simulink model "turbo_controller"  (R2025a)
settings: Solver=FixedStepAuto  StartTime=0.0  StopTime=inf  FixedStep=0.001  RelTol=1e-3
PostLoadFcn:
  | % 自动定位同目录CubeMX文件；不需要外部初始化脚本。
  | codertarget.data.setParameterValue('turbo_controller','STM32CubeMX.ProjectFile',fullfile(fileparts(get_param('turbo_controller','FileName')),'turbo_f407.ioc'));
InitFcn:
  | % 中文说明：按原控制器字段与类型创建三组接口总线；控制参数已内嵌。
  | tc_names=["EValve_Cycle" "EValve_Open" "Eblast_Cycle" "Eblast_Open" "Motor_Cycle" "Motor_Open" "EValve_Enable" "Eblast_Enable" "Motor_Enable" "SWO_Firework" "SWO_BleedAir" "EngineState" "Flag_ECUReset_Clear" "Flag_ECUReset_Save" "Flag_Reset_Enable" "Accelerator" "Nc_dem" "Nc"]; tc_types=["uint16" "uint16" "uint16" "uint16" "uint16" "uint16" "uint8" "uint8" "uint8" "uint8" "uint8" "uint8" "uint8" "uint8" "uint8" "single" "single" "single"];
  | for tc_k=1:numel(tc_names)
  |  tc_e(tc_k)=Simulink.BusElement; tc_e(tc_k).Name=char(tc_names(tc_k)); tc_e(tc_k).DataType=char(tc_types(tc_k));
  | end
  | EngineControl_Out=Simulink.Bus; EngineControl_Out.DataScope='Exported'; EngineControl_Out.Elements=tc_e;
  | clear tc_e tc_names tc_types tc_k
  | tc_names=["savedata1" "savedata2" "savedata3" "savedata4" "savedata5" "savedata6" "savedata7" "savedata8" "savedata9" "savedata10" "savedata11" "savedata12" "savedata13" "savedata14" "savedata15" "savedata16" "savedata17" "savedata18" "savedata19" "savedata20" "savedata21" "savedata22" "savedata23" "savedata24" "savedata25"]; tc_types=["single" "single" "single" "single" "single" "single" "single" "single" "single" "single" "single" "single" "single" "single" "single" "single" "single" "single" "single" "single" "single" "single" "single" "single" "single"];
  | for tc_k=1:numel(tc_names)
  |  tc_e(tc_k)=Simulink.BusElement; tc_e(tc_k).Name=char(tc_names(tc_k)); tc_e(tc_k).DataType=char(tc_types(tc_k));
  | end
  | SaveData_Out=Simulink.Bus; SaveData_Out.DataScope='Exported'; SaveData_Out.Elements=tc_e;
  | clear tc_e tc_names tc_types tc_k
  | tc_names=["senddata1" "senddata2" "senddata3" "senddata4" "senddata5" "senddata6" "senddata7" "senddata8" "senddata9" "senddata10" "senddata11" "senddata12" "senddata13" "senddata14" "senddata15" "senddata16" "senddata17" "senddata18" "senddata19" "senddata20" "senddata21" "senddata22" "senddata23" "senddata24" "senddata25" "senddata26" "senddata27" "senddata28" "senddata29"]; tc_types=["uint8" "uint8" "uint8" "uint8" "uint8" "uint8" "uint8" "uint8" "uint8" "uint8" "uint8" "uint8" "uint8" "uint8" "uint8" "uint8" "uint8" "uint8" "uint8" "uint8" "uint8" "uint8" "uint8" "uint8" "uint8" "uint8" "uint8" "uint8" "uint8"];
  | for tc_k=1:numel(tc_names)
  |  tc_e(tc_k)=Simulink.BusElement; tc_e(tc_k).Name=char(tc_names(tc_k)); tc_e(tc_k).DataType=char(tc_types(tc_k));
  | end
  | SendData_Out=Simulink.Bus; SendData_Out.DataScope='Exported'; SendData_Out.Elements=tc_e;
  | clear tc_e tc_names tc_types tc_k
  | 
  | % 以下为接口中文说明；只设置描述，不改变数值或数据类型。
  | EngineControl_Out.Description='执行控制输出（阀、电机、点火、状态及复位请求）';
  | tc_cn=["EValve_Cycle（主油阀周期计数（每计数2毫秒））" "EValve_Open（主油阀开通计数（每计数2毫秒））" "Eblast_Cycle（副油阀周期计数（每计数2毫秒））" "Eblast_Open（副油阀开通计数（每计数2毫秒））" "Motor_Cycle（起动电机周期计数）" "Motor_Open（起动电机开通计数）" "EValve_Enable（主油阀驱动使能）" "Eblast_Enable（副油阀驱动使能）" "Motor_Enable（起动电机使能）" "SWO_Firework（点火器使能（1开））" "SWO_BleedAir（引气阀使能（1开））" "EngineState（发动机状态）" "Flag_ECUReset_Clear（清除复位恢复状态请求）" "Flag_ECUReset_Save（保存复位恢复数据请求）" "Flag_Reset_Enable（处理器软件复位请求）" "Accelerator（油门／油泵给定控制量）" "Nc_dem（控制目标转速）" "Nc（发动机反馈转速（转每分））"];
  | tc_elements=EngineControl_Out.Elements;
  | for tc_k=1:numel(tc_cn)
  |  tc_elements(tc_k).Description=char(tc_cn(tc_k));
  | end
  | EngineControl_Out.Elements=tc_elements;
  | clear tc_cn tc_elements tc_k
  | SaveData_Out.Description='25项运行记录；字段含义按当前模型数据来源解释';
  | tc_cn=["savedata1（指令回显记录）" "savedata2（入口总温记录（℃））" "savedata3（电源电压记录）" "savedata4（排气温度记录（℃））" "savedata5（标定燃油压力记录）" "savedata6（副油阀占空比记录（％））" "savedata7（主油阀占空比记录（％））" "savedata8（温度修正转速记录）" "savedata9（开关输出及反馈位域）" "savedata10（物理转速记录）" "savedata11（油泵目标给定原始值）" "savedata12（起动电机占空比记录（％））" "savedata13（发动机状态码记录）" "savedata14（故障告警位域记录）" "savedata15（模型记录帧序号）" "savedata16（处理器温度记录（℃））" "savedata17（装订转速记录（沿用旧电源字段名））" "savedata18（导航高度记录）" "savedata19（飞行空速记录）" "savedata20（主阀旧记录位（恒零保留））" "savedata21（第21项保留记录（恒零））" "savedata22（保留记录项22）" "savedata23（保留记录项23）" "savedata24（保留记录项24）" "savedata25（保留记录项25）"];
  | tc_elements=SaveData_Out.Elements;
  | for tc_k=1:numel(tc_cn)
  |  tc_elements(tc_k).Description=char(tc_cn(tc_k));
  | end
  | SaveData_Out.Elements=tc_elements;
  | clear tc_cn tc_elements tc_k
  | SendData_Out.Description='29字段回传及外设命令接口；板端上位机帧只取第3至27字段';
  | tc_cn=["senddata1（回传发送允许标志（不直接上线路））" "senddata2（回传载荷长度25字节）" "senddata3（回传指令回显字节）" "senddata4（总温编码字节（℃＋80））" "senddata5（电源电压编码字节）" "senddata6（排温编码高字节）" "senddata7（排温编码低字节）" "senddata8（燃油压力编码高字节）" "senddata9（燃油压力编码低字节）" "senddata10（副油阀占空比字节（％））" "senddata11（主油阀占空比字节（％））" "senddata12（修正转速编码高字节）" "senddata13（修正转速编码低字节）" "senddata14（驱动及反馈状态位域）" "senddata15（物理转速编码高字节）" "senddata16（物理转速编码低字节）" "senddata17（油泵目标给定高字节（串口二使用））" "senddata18（油泵目标给定低字节（串口二使用））" "senddata19（起动电机占空比命令（串口一使用））" "senddata20（发动机状态码字节）" "senddata21（故障告警位域字节）" "senddata22（帧序号占位（板端另行填写））" "senddata23（处理器温度编码（℃＋50））" "senddata24（控制目标转速编码高字节）" "senddata25（控制目标转速编码低字节）" "senddata26（占位字节（板端改填实测泵速高字节））" "senddata27（占位字节（板端改填实测泵速低字节））" "senddata28（装订转速高字节（本板未发送））" "senddata29（装订转速低字节（本板未发送））"];
  | tc_elements=SendData_Out.Elements;
  | for tc_k=1:numel(tc_cn)
  |  tc_elements(tc_k).Description=char(tc_cn(tc_k));
  | end
  | SendData_Out.Elements=tc_elements;
  | clear tc_cn tc_elements tc_k
  | 
  | 
  | % FRAM模块化事务：接口类型和上电初始状态，随模型保存，无外部初始化文件。
  | clear FM_elements
  | FM_elements(1)=Simulink.BusElement;FM_elements(1).Name='phase';FM_elements(1).DataType='uint8';FM_elements(1).Dimensions=[1 1];FM_elements(1).Description='phase（当前事务阶段）';
  | FM_elements(2)=Simulink.BusElement;FM_elements(2).Name='a';FM_elements(2).DataType='uint8';FM_elements(2).Dimensions=[64 1];FM_elements(2).Description='a（启动时缓存的首区64字节）';
  | FM_elements(3)=Simulink.BusElement;FM_elements(3).Name='active';FM_elements(3).DataType='uint16';FM_elements(3).Dimensions=[1 1];FM_elements(3).Description='active（当前有效记录区地址）';
  | FM_elements(4)=Simulink.BusElement;FM_elements(4).Name='generation';FM_elements(4).DataType='uint32';FM_elements(4).Dimensions=[1 1];FM_elements(4).Description='generation（当前有效记录代号）';
  | FM_elements(5)=Simulink.BusElement;FM_elements(5).Name='record';FM_elements(5).DataType='uint8';FM_elements(5).Dimensions=[64 1];FM_elements(5).Description='record（本次冻结的待写记录）';
  | FM_elements(6)=Simulink.BusElement;FM_elements(6).Name='addr';FM_elements(6).DataType='uint16';FM_elements(6).Dimensions=[1 1];FM_elements(6).Description='addr（本次备用写入地址）';
  | FM_elements(7)=Simulink.BusElement;FM_elements(7).Name='lastSave';FM_elements(7).DataType='single';FM_elements(7).Dimensions=[1 1];FM_elements(7).Description='lastSave（上次开始保存的秒数）';
  | FM_elements(8)=Simulink.BusElement;FM_elements(8).Name='lastState';FM_elements(8).DataType='uint8';FM_elements(8).Dimensions=[1 1];FM_elements(8).Description='lastState（上次保存时的发动机状态）';
  | FM_elements(9)=Simulink.BusElement;FM_elements(9).Name='boot';FM_elements(9).DataType='boolean';FM_elements(9).Dimensions=[1 1];FM_elements(9).Description='boot（启动记录是否允许恢复）';
  | FM_elements(10)=Simulink.BusElement;FM_elements(10).Name='consumed';FM_elements(10).DataType='boolean';FM_elements(10).Dimensions=[1 1];FM_elements(10).Description='consumed（本次启动恢复通知是否已发送）';
  | FM_elements(11)=Simulink.BusElement;FM_elements(11).Name='payload';FM_elements(11).DataType='uint8';FM_elements(11).Dimensions=[20 1];FM_elements(11).Description='payload（当前20字节恢复内容）';
  | ... (+35 lines)
model workspace (MAT data in the model file):
  CRC16_Table_Reference = [0 4129 8258 12387 16516 20645 24774 28903 33032 37161 41290 45419 ... (256 elements, 256x1)]
  PE_Kaer = [0.15402 0.15402 0.12264 0.10076 0.09481 0.07601 0.07111 0.0569 0.05198 0.04926 0.05308 0.04325 ... (13 elements, 1x13)]
  PE_Nr = [21.2982 61.4260372 67.7475458 72.7394382 76.845934 80.6988798 83.8449282 86.6491912 88.9382406 89.178606 91.1938214 93.4068058 ... (13 elements, 1x13)]
  PE_Pump_Translate = 33.5999984741
  PE_RotaSpeed_Translate = 860
  PE_Taer = [0.4939154 0.4939154 0.40780982 0.34066978 0.31622756 0.30405716 0.34300244 0.26785022 0.37393554 0.23914836 0.44563948 0.31044662 ... (13 elements, 1x13)]
  PF_ACCFULLRANGE = 3360
  PF_Flag_ECUReset = 0
  PF_Flag_rx_suc = 1
  PF_Gear_Info = [40000; 45000; 50000; 55000; 57000; 59000; 60000; 61000; 61000; 61000; 61000; 61000]
  PF_K_TiaoJie = 1
  PF_Kpu = 10
  PF_MySet_Rxdata = [0 0 0 0 0 0 0 0 0 0 0 0 ... (50 elements, 50x1)]
  PF_MyUsart1_Rxdata = [0 0 0 0 0 0 0 0 0 0 0 0 ... (50 elements, 50x1)]
  PF_MyUsart2_Rxdata = [0 0 0 0 0 0 0 0 0 0 0 0 ... (50 elements, 50x1)]
  PF_Reset_Information = [0 0 0 0 0 0 0 0 0 0 0 0 ... (20 elements, 20x1)]
  PF_Sensor_X1_T4 = [0 4095]
  PF_Sensor_X2_T4 = [0 1.66666698456]
  PF_Sensor_X3_T4 = [0 504 999 1497 2010 2529 3051 3568 4076 4571 4959]
  PF_Sensor_X_P2 = [0.5 3]
  PF_Sensor_X_Poil = [0.5 3]
  PF_Sensor_X_T1t = [-50 300]
  PF_Sensor_X_Vpower = [0 3]
  PF_Sensor_X_Vpump = [0 3]
  PF_Sensor_Y1_T4 = [0 3]
  PF_Sensor_Y2_T4 = [0 5000]
  PF_Sensor_Y3_T4 = [0 100 200 300 400 500 600 700 800 900 980]
  PF_Sensor_Y_P2 = [0 1000]
  PF_Sensor_Y_Poil = [0 1000]
  PF_Sensor_Y_T1t = [-50 300]
  PF_Sensor_Y_Vpower = [0 33]
  PF_Sensor_Y_Vpump = [0 33]
  PG_CtrlMode_CloseLoop : mpt.Parameter (value not decoded)
  PG_CtrlMode_ManualAcc : mpt.Parameter (value not decoded)
  PG_CtrlMode_Origin : mpt.Parameter (value not decoded)
  PG_CtrlMode_Start : mpt.Parameter (value not decoded)
  PG_CtrlMode_Stop : mpt.Parameter (value not decoded)
  PG_ES_Clp : mpt.Parameter (value not decoded)
  PG_ES_EngStart : mpt.Parameter (value not decoded)
  PG_ES_Manual : mpt.Parameter (value not decoded)
  PG_ES_Origin : mpt.Parameter (value not decoded)
  PG_ES_Stop : mpt.Parameter (value not decoded)
  PG_Instr_BleedAirSet : mpt.Parameter (value not decoded)
  PG_Instr_CloseLoop : mpt.Parameter (value not decoded)
  PG_Instr_ECUReSet : mpt.Parameter (value not decoded)
  PG_Instr_EValveSet : mpt.Parameter (value not decoded)
  PG_Instr_EblastSet : mpt.Parameter (value not decoded)
  PG_Instr_Erase : mpt.Parameter (value not decoded)
  PG_Instr_FireWorkSet : mpt.Parameter (value not decoded)
  PG_Instr_ManualPlus : mpt.Parameter (value not decoded)
  PG_Instr_ManualrReduce : mpt.Parameter (value not decoded)
  PG_Instr_MotorSet : mpt.Parameter (value not decoded)
  PG_Instr_OilSet : mpt.Parameter (value not decoded)
  PG_Instr_SelfCheck : mpt.Parameter (value not decoded)
  PG_Instr_Start : mpt.Parameter (value not decoded)
  PG_Instr_Stop : mpt.Parameter (value not decoded)
  PG_Instr_StopZero : Simulink.Parameter (value not decoded)
  PG_Location_Air : Simulink.Parameter (value not decoded)
  PG_Location_Gnd : Simulink.Parameter (value not decoded)
  PG_ServoCtrlMode_CloseLoop : Simulink.Parameter (value not decoded)
  PG_ServoCtrlMode_CloseLoopMax : Simulink.Parameter (value not decoded)
  PG_ServoCtrlMode_CloseLoopMin : Simulink.Parameter (value not decoded)
  PG_ServoCtrlMode_ManualAcc : Simulink.Parameter (value not decoded)
  PG_ServoCtrlMode_ManualAccMax : Simulink.Parameter (value not decoded)
  PG_ServoCtrlMode_ManualAccMin : Simulink.Parameter (value not decoded)
  PG_SpeedDot_Permit : Simulink.Parameter (value not decoded)
  PL_EngineModel_Actuator = [0 10 100]
  PL_EngineModel_EngineStar_Press_P2 = [1013 1098.4 1099.144828 1099.931034 1103.613793 1162.662069 1143.793103 1131.006897 1123.186207 1117.6 1114 1111.806897 ... (127 elements, 1x127)]
  PL_EngineModel_EngineStar_RotaSpeed = [200 2000 9584 9660 10220 10240 10260 10288 10308 10368 10380 10408 ... (127 elements, 1x127)]
  PL_EngineModel_EngineStar_Temp_Exhaust = [128 129 129.1 130 131 131.1 132 133 134 134.1 135 135.1 ... (127 elements, 1x127)]
  PL_EngineModel_EngineStar_Time = [0.05 0.1 0.15 0.2 0.25 0.3 0.35 0.4 0.45 0.5 0.55 0.6 ... (127 elements, 1x127)]
  PL_EngineModel_IdleAbove_Nr = [0 21.2982 61.4260372 67.7475458 72.7394382 76.845934 80.6988798 83.8449282 86.6491912 88.9382406 89.178606 91.1938214 ... (14 elements, 1x14)]
  PL_EngineModel_IdleAbove_P2r = [0.986923266716 1.57907722675 1.81593881076 1.99358499877 2.23044658278 2.43770046879 2.65482358747 2.84233900814 3.03972366149 3.18776215149 3.25684678016 3.3950160375 ... (14 elements, 1x14)]
  PL_EngineModel_IdleAbove_Tempr = [0.0536001429337 1.07200285867 1.63301768805 1.63659103091 1.66875111667 1.72592460247 1.77595140254 1.86171163123 1.95461854565 2.03323208862 2.03323208862 2.13685903162 ... (14 elements, 1x14)]
  PL_EngineModel_IdleAbove_Ter = [0.42434128 0.42434128 0.42434128 0.30669408 0.23570008 0.22150128 0.1997974 0.23803274 0.16115638 0.24279948 0.13600422 0.31308354 ... (14 elements, 1x14)]
  PL_EngineModel_IdleAbove_Wfr = [0 10.142 23.8337 27.8905 31.9473 36.0041 40.0609 44.1177 48.1745 52.2313 52.7384 56.7952 ... (14 elements, 1x14)]
  PL_EngineModel_Press_P2 = [400 400 400 400 400 400 400 400 400 400]
  PL_EngineModel_Rotaspeed = [0 20000 96400]
  PL_EngineModel_Temp_Exhaust = [500 500 500 500 500 500 500 500 500 500]
  PL_Kaer = [0.1 0.1 0.1 0.1 0.1 0.1]
  PL_Nr = [50 60 70 80 90 100]
  PL_Taer = [0.1 0.1 0.1 0.1 0.1 0.1]
  Sig : Simulink.Signal (value not decoded)
  Ts_ms : Simulink.Parameter (value not decoded)
  false : Simulink.Parameter (value not decoded)
  true : Simulink.Parameter (value not decoded)
symbols that are objects in the model workspace (value not decoded): PG_CtrlMode_CloseLoop, PG_CtrlMode_ManualAcc, PG_CtrlMode_Origin, PG_CtrlMode_Start, PG_CtrlMode_Stop, PG_ES_Clp, PG_ES_EngStart, PG_ES_Manual, PG_ES_Origin, PG_ES_Stop, PG_Instr_BleedAirSet, PG_Instr_CloseLoop, PG_Instr_EblastSet, PG_Instr_ECUReSet, PG_Instr_Erase, PG_Instr_EValveSet, PG_Instr_FireWorkSet, PG_Instr_ManualPlus, PG_Instr_ManualrReduce, PG_Instr_MotorSet, PG_Instr_OilSet, PG_Instr_SelfCheck, PG_Instr_Start, PG_Instr_Stop, PG_Instr_StopZero, PG_ServoCtrlMode_CloseLoop, PG_ServoCtrlMode_CloseLoopMax, PG_ServoCtrlMode_CloseLoopMin, PG_ServoCtrlMode_ManualAcc, PG_ServoCtrlMode_ManualAccMax, PG_ServoCtrlMode_ManualAccMin, Ts_ms
libraries: simulink x97, stm32blockslib x10, stm32f4xxblockslib x8
(part 17 of 26)

== system turbo_controller/ESM/Flags/EngineStop ==
  note: 【本页库子系统中文说明】TingCheZhiLing
      | 一、它做什么？
      | 这是“过不过这条线”的判断器。将输入与阈值 PG_Instr_Stop 作 == 比较，关系成
      | 立输出真（1），否则输出假（0）。例如>=包含恰好等于，>则不包含。它只给出判断
      | 标志，不会自行限幅、报警、切换状态或操作阀门；后续逻辑决定如何使用。名称可能
      | 只是用途提示，实际判据以这里的关系和阈值为准。
      | 二、本实例当前参数
      | 比较关系：==
      | 比较阈值：PG_Instr_Stop
      | 输出数据类型：布尔值，真或假
      | 零交叉检测：开启
      | 三、怎样继续学习？
      | 这是标准库子系统实例。中文说明放在使用它的父级页面，并同步存入本块Descriptio
      | n（模块说明）；官方库链接保留。先看本实例的输入来自哪里、输出交给谁，再结合
      | 以上参数理解作用。
  note: 【本页库子系统中文说明】TingCheZhiLing1
      | 一、它做什么？
      | 这是“过不过这条线”的判断器。将输入与阈值 PG_Instr_StopZero 作 == 比较，关
      | 系成立输出真（1），否则输出假（0）。例如>=包含恰好等于，>则不包含。它只给出
      | 判断标志，不会自行限幅、报警、切换状态或操作阀门；后续逻辑决定如何使用。名称
      | 可能只是用途提示，实际判据以这里的关系和阈值为准。
      | 二、本实例当前参数
      | 比较关系：==
      | 比较阈值：PG_Instr_StopZero
      | 输出数据类型：布尔值，真或假
      | 零交叉检测：开启
      | 三、怎样继续学习？
      | 这是标准库子系统实例。中文说明放在使用它的父级页面，并同步存入本块Descriptio
      | n（模块说明）；官方库链接保留。先看本实例的输入来自哪里、输出交给谁，再结合
      | 以上参数理解作用。
  note: 把停车命令和起动异常转换成停车请求
      |
      | Stop和StopZero命令都可形成相应停车转换条件；起动内部阶段结果4或15也参与起动转停车判断，用
      | 于流程异常或退出。
      |
      | 分别输出Clp2Stop、Manual2Stop、Start2Stop，交状态机按当前模式选择。内部阶段结果15并不是对
      | 外EngineState=15；对外停车模式编号仍为4。
      |
      | 本模块只提出转换要求，停车后关闭油路、是否短时拖转及何时完成由Stop分支处理。
  note: Compare
      | To Constant1
      | CompareTo Constant1：只判断一个条件
      |
      | 把输入与4比较，使用关系“==”。成立输出1，不成立输出0；输出是判断标志，不是把输入缩放成该
      | 常数。
      |
      | 比较门限用于父级的分支条件，没有滤波、延时确认或锁存。例如输入恰好等于门限时，“>=、<=、==
      | ”成立，“>、<”不成立。是否需要持续确认或同时满足其他条件，由父级连线决定。
  note: Compare
      | To Constant2
      | CompareTo Constant2：只判断一个条件
      |
      | 把输入与15比较，使用关系“==”。成立输出1，不成立输出0；输出是判断标志，不是把输入缩放成该
      | 常数。
      |
      | 比较门限用于父级的分支条件，没有滤波、延时确认或锁存。例如输入恰好等于门限时，“>=、<=、==
      | ”成立，“>、<”不成立。是否需要持续确认或同时满足其他条件，由父级连线决定。
  note: TingCheZhiLing
      | TingCheZhiLing：只判断一个条件
      |
      | 把输入与6比较，使用关系“==”。成立输出1，不成立输出0；输出是判断标志，不是把输入缩放成该
      | 常数。
      |
      | 这里识别一种指令编码。判断成立只说明指令匹配；父级还会结合有效帧、当前模式或其他允许条件决
      | 定是否更新。实际驱动要继续经过控制与板级输出，不能把1理解为硬件执行回执。
  note: TingCheZhiLing1
      | TingCheZhiLing1：只判断一个条件
      |
      | 把输入与15比较，使用关系“==”。成立输出1，不成立输出0；输出是判断标志，不是把输入缩放成该
      | 常数。
      |
      | 这里识别一种指令编码。判断成立只说明指令匹配；父级还会结合有效帧、当前模式或其他允许条件决
      | 定是否更新。实际驱动要继续经过控制与板级输出，不能把1理解为硬件执行回执。
  S_Flag_EnigneState : Inport
      settings: AttributesFormatString=S_Flag_EnigneState（发动机状态标志）
  S_Instr : Inport  Port=2
      settings: AttributesFormatString=S_Instr（指令）
  Compare To Constant1 : simulink/Logic and Bit Operations/Compare To Constant  Description=|  relop===  const=4  OutDataTypeStr=boolean
      | CompareTo Constant1：只判断一个条件
      | 
      | 把输入与4比较，使用关系“==”。成立输出1，不成立输出0；输出是判断标志，不是把输入缩放成该常数。
      | 
      | 比较门限用于父级的分支条件，没有滤波、延时确认或锁存。例如输入恰好等于门限时，“>=、<=、==”成立，“>、<”不成立。是否需要持续确认或同时满足其他条件，由父级连线决定。
      settings: AttributesFormatString=Compare To Constant1（比较到常量1）
  Compare To Constant2 : simulink/Logic and Bit Operations/Compare To Constant  Description=|  relop===  const=15  OutDataTypeStr=boolean
      | CompareTo Constant2：只判断一个条件
      | 
      | 把输入与15比较，使用关系“==”。成立输出1，不成立输出0；输出是判断标志，不是把输入缩放成该常数。
      | 
      | 比较门限用于父级的分支条件，没有滤波、延时确认或锁存。例如输入恰好等于门限时，“>=、<=、==”成立，“>、<”不成立。是否需要持续确认或同时满足其他条件，由父级连线决定。
      settings: AttributesFormatString=Compare To Constant2（比较到常量2）
  Constant1 : Constant  Value=true  OutDataTypeStr=boolean  SampleTime=-1
      settings: AttributesFormatString=Constant1（常量1）
  Constant13 : Constant  Value=false  OutDataTypeStr=boolean  SampleTime=-1
      settings: AttributesFormatString=Constant13（常量13）
  Logical Operator : Logic  Operator=OR  Inputs=3  AllPortsSameDT=off  OutDataTypeStr=boolean
      settings: AttributesFormatString=Logical Operator（逻辑运算）
  Logical Operator1 : Logic  Operator=OR  AllPortsSameDT=off  OutDataTypeStr=boolean
      settings: AttributesFormatString=Logical Operator1（逻辑运算1）
  Switch : Switch  Criteria=u2 ~= 0  SaturateOnIntegerOverflow=off  InputSameDT=off
      settings: AttributesFormatString=Switch（开关选择）
  TingCheZhiLing : simulink/Logic and Bit Operations/Compare To Constant  Description=|  relop===  const=PG_Instr_Stop  OutDataTypeStr=boolean
      | TingCheZhiLing：只判断一个条件
      | 
      | 把输入与6比较，使用关系“==”。成立输出1，不成立输出0；输出是判断标志，不是把输入缩放成该常数。
      | 
      | 这里识别一种指令编码。判断成立只说明指令匹配；父级还会结合有效帧、当前模式或其他允许条件决定是否更新。实际驱动要继续经过控制与板级输出，不能把1理解为硬件执行回执。
      settings: AttributesFormatString=TingCheZhiLing（停车指令）
  TingCheZhiLing1 : simulink/Logic and Bit Operations/Compare To Constant  Description=|  relop===  const=PG_Instr_StopZero  OutDataTypeStr=boolean
      | TingCheZhiLing1：只判断一个条件
      | 
      | 把输入与15比较，使用关系“==”。成立输出1，不成立输出0；输出是判断标志，不是把输入缩放成该常数。
      | 
      | 这里识别一种指令编码。判断成立只说明指令匹配；父级还会结合有效帧、当前模式或其他允许条件决定是否更新。实际驱动要继续经过控制与板级输出，不能把1理解为硬件执行回执。
      settings: AttributesFormatString=TingCheZhiLing1（停车指令1）
  S_Clp2Stop : Outport
      settings: AttributesFormatString=S_Clp2Stop（闭环转停车）
  S_Manual2Stop : Outport  Port=2
      settings: AttributesFormatString=S_Manual2Stop（手动转停车）
  S_Start2Stop : Outport  Port=3
      settings: AttributesFormatString=S_Start2Stop（起动转停车）
  wires:
  Constant13/1 -> Switch/3
  Constant1/1 -> Switch/1
  Switch/1 -> S_Manual2Stop/1, Logical Operator/1, S_Clp2Stop/1
  S_Instr/1 -> TingCheZhiLing1/1, TingCheZhiLing/1
  S_Flag_EnigneState/1 -> Compare To Constant1/1, Compare To Constant2/1
  Compare To Constant1/1 -> Logical Operator/2
  Logical Operator/1 -> S_Start2Stop/1
  Compare To Constant2/1 -> Logical Operator/3
  TingCheZhiLing1/1 -> Logical Operator1/2
  TingCheZhiLing/1 -> Logical Operator1/1
  Logical Operator1/1 -> Switch/2

== system turbo_controller/ESM/Flags/Manual ==
  note: 【本页库子系统中文说明】ShouDongBeiFa
      | 一、它做什么？
      | 这是“过不过这条线”的判断器。将输入与阈值 PG_Instr_EblastSet 作 == 比较，关
      | 系成立输出真（1），否则输出假（0）。例如>=包含恰好等于，>则不包含。它只给出
      | 判断标志，不会自行限幅、报警、切换状态或操作阀门；后续逻辑决定如何使用。名称
      | 可能只是用途提示，实际判据以这里的关系和阈值为准。
      | 二、本实例当前参数
      | 比较关系：==
      | 比较阈值：PG_Instr_EblastSet
      | 输出数据类型：布尔值，真或假
      | 零交叉检测：开启
      | 三、怎样继续学习？
      | 这是标准库子系统实例。中文说明放在使用它的父级页面，并同步存入本块Descriptio
      | n（模块说明）；官方库链接保留。先看本实例的输入来自哪里、输出交给谁，再结合
      | 以上参数理解作用。
  note: 【本页库子系统中文说明】ShouDongDianHuo
      | 一、它做什么？
      | 这是“过不过这条线”的判断器。将输入与阈值 PG_Instr_FireWorkSet 作 == 比较，
      | 关系成立输出真（1），否则输出假（0）。例如>=包含恰好等于，>则不包含。它只给
      | 出判断标志，不会自行限幅、报警、切换状态或操作阀门；后续逻辑决定如何使用。名
      | 称可能只是用途提示，实际判据以这里的关系和阈值为准。
      | 二、本实例当前参数
      | 比较关系：==
      | 比较阈值：PG_Instr_FireWorkSet
      | 输出数据类型：布尔值，真或假
      | 零交叉检测：开启
      | 三、怎样继续学习？
      | 这是标准库子系统实例。中文说明放在使用它的父级页面，并同步存入本块Descriptio
      | n（模块说明）；官方库链接保留。先看本实例的输入来自哪里、输出交给谁，再结合
      | 以上参数理解作用。
  note: 【本页库子系统中文说明】ShouDongDianJi
      | 一、它做什么？
      | 这是“过不过这条线”的判断器。将输入与阈值 PG_Instr_MotorSet 作 == 比较，关
      | 系成立输出真（1），否则输出假（0）。例如>=包含恰好等于，>则不包含。它只给出
      | 判断标志，不会自行限幅、报警、切换状态或操作阀门；后续逻辑决定如何使用。名称
      | 可能只是用途提示，实际判据以这里的关系和阈值为准。
      | 二、本实例当前参数
      | 比较关系：==
      | 比较阈值：PG_Instr_MotorSet
      | 输出数据类型：布尔值，真或假
      | 零交叉检测：开启
      | 三、怎样继续学习？
      | 这是标准库子系统实例。中文说明放在使用它的父级页面，并同步存入本块Descriptio
      | n（模块说明）；官方库链接保留。先看本实例的输入来自哪里、输出交给谁，再结合
      | 以上参数理解作用。
  note: 【本页库子系统中文说明】ShouDongJia
      | 一、它做什么？
      | 这是“过不过这条线”的判断器。将输入与阈值 PG_Instr_ManualPlus 作 == 比较，
      | 关系成立输出真（1），否则输出假（0）。例如>=包含恰好等于，>则不包含。它只给
      | 出判断标志，不会自行限幅、报警、切换状态或操作阀门；后续逻辑决定如何使用。名
      | 称可能只是用途提示，实际判据以这里的关系和阈值为准。
      | 二、本实例当前参数
      | 比较关系：==
      | 比较阈值：PG_Instr_ManualPlus
      | 输出数据类型：布尔值，真或假
      | 零交叉检测：开启
      | 三、怎样继续学习？
      | 这是标准库子系统实例。中文说明放在使用它的父级页面，并同步存入本块Descriptio
      | n（模块说明）；官方库链接保留。先看本实例的输入来自哪里、输出交给谁，再结合
      | 以上参数理解作用。
  note: 【本页库子系统中文说明】ShouDongJian
      | 一、它做什么？
      | 这是“过不过这条线”的判断器。将输入与阈值 PG_Instr_ManualrReduce 作 == 比较
      | ，关系成立输出真（1），否则输出假（0）。例如>=包含恰好等于，>则不包含。它只
      | 给出判断标志，不会自行限幅、报警、切换状态或操作阀门；后续逻辑决定如何使用。
      | 名称可能只是用途提示，实际判据以这里的关系和阈值为准。
      | 二、本实例当前参数
      | 比较关系：==
      | 比较阈值：PG_Instr_ManualrReduce
      | 输出数据类型：布尔值，真或假
      | 零交叉检测：开启
      | 三、怎样继续学习？
      | 这是标准库子系统实例。中文说明放在使用它的父级页面，并同步存入本块Descriptio
      | n（模块说明）；官方库链接保留。先看本实例的输入来自哪里、输出交给谁，再结合
      | 以上参数理解作用。
  note: 【本页库子系统中文说明】ShouDongYinQi
      | 一、它做什么？
      | 这是“过不过这条线”的判断器。将输入与阈值 PG_Instr_BleedAirSet 作 == 比较，
      | 关系成立输出真（1），否则输出假（0）。例如>=包含恰好等于，>则不包含。它只给
      | 出判断标志，不会自行限幅、报警、切换状态或操作阀门；后续逻辑决定如何使用。名
      | 称可能只是用途提示，实际判据以这里的关系和阈值为准。
      | 二、本实例当前参数
      | 比较关系：==
      | 比较阈值：PG_Instr_BleedAirSet
      | 输出数据类型：布尔值，真或假
      | 零交叉检测：开启
      | 三、怎样继续学习？
      | 这是标准库子系统实例。中文说明放在使用它的父级页面，并同步存入本块Descriptio
      | n（模块说明）；官方库链接保留。先看本实例的输入来自哪里、输出交给谁，再结合
      | 以上参数理解作用。
  note: 【本页库子系统中文说明】ShouDongYouMen
      | 一、它做什么？
      | 这是“过不过这条线”的判断器。将输入与阈值 PG_Instr_OilSet 作 == 比较，关系
      | 成立输出真（1），否则输出假（0）。例如>=包含恰好等于，>则不包含。它只给出判
      | 断标志，不会自行限幅、报警、切换状态或操作阀门；后续逻辑决定如何使用。名称可
      | 能只是用途提示，实际判据以这里的关系和阈值为准。
      | 二、本实例当前参数
      | 比较关系：==
      | 比较阈值：PG_Instr_OilSet
      | 输出数据类型：布尔值，真或假
      | 零交叉检测：开启
      | 三、怎样继续学习？
      | 这是标准库子系统实例。中文说明放在使用它的父级页面，并同步存入本块Descriptio
      | n（模块说明）；官方库链接保留。先看本实例的输入来自哪里、输出交给谁，再结合
      | 以上参数理解作用。
  note: 【本页库子系统中文说明】ShouDongZhuFa
      | 一、它做什么？
      | 这是“过不过这条线”的判断器。将输入与阈值 PG_Instr_EValveSet 作 == 比较，关
      | 系成立输出真（1），否则输出假（0）。例如>=包含恰好等于，>则不包含。它只给出
      | 判断标志，不会自行限幅、报警、切换状态或操作阀门；后续逻辑决定如何使用。名称
      | 可能只是用途提示，实际判据以这里的关系和阈值为准。
      | 二、本实例当前参数
      | 比较关系：==
      | 比较阈值：PG_Instr_EValveSet
      | 输出数据类型：布尔值，真或假
      | 零交叉检测：开启
      | 三、怎样继续学习？
      | 这是标准库子系统实例。中文说明放在使用它的父级页面，并同步存入本块Descriptio
      | n（模块说明）；官方库链接保留。先看本实例的输入来自哪里、输出交给谁，再结合
      | 以上参数理解作用。
  note: 识别会进入手动模式的八类命令
      |
      | 比较当前命令是否属于手动泵直接设定、加、减、主油阀、副油阀、起动电机、点火器或引气阀设置。
      | 任一匹配便形成进入手动的条件。
      |
      | 分别向初始、起动、闭环模式提供转Manual标志，真正能用哪一条由状态机的当前状态决定。这里不解
      | 释Data6的开度和数值；进入手动后，CLM/Manual才把命令参数换成具体执行器设定。
  note: ShouDongBeiFa
      | ShouDongBeiFa：只判断一个条件
      |
      | 把输入与12比较，使用关系“==”。成立输出1，不成立输出0；输出是判断标志，不是把输入缩放成该
      | 常数。
      |
      | 这里识别一种指令编码。判断成立只说明指令匹配；父级还会结合有效帧、当前模式或其他允许条件决
      | 定是否更新。实际驱动要继续经过控制与板级输出，不能把1理解为硬件执行回执。
  note: ShouDongDianHuo
      | ShouDongDianHuo：只判断一个条件
      |
      | 把输入与10比较，使用关系“==”。成立输出1，不成立输出0；输出是判断标志，不是把输入缩放成该
      | 常数。
      |
      | 这里识别一种指令编码。判断成立只说明指令匹配；父级还会结合有效帧、当前模式或其他允许条件决
      | 定是否更新。实际驱动要继续经过控制与板级输出，不能把1理解为硬件执行回执。
  note: ShouDongDianJi
      | ShouDongDianJi：只判断一个条件
      |
      | 把输入与13比较，使用关系“==”。成立输出1，不成立输出0；输出是判断标志，不是把输入缩放成该
      | 常数。
      |
      | 这里识别一种指令编码。判断成立只说明指令匹配；父级还会结合有效帧、当前模式或其他允许条件决
      | 定是否更新。实际驱动要继续经过控制与板级输出，不能把1理解为硬件执行回执。
  note: ShouDongJia
      | ShouDongJia：只判断一个条件
      |
      | 把输入与4比较，使用关系“==”。成立输出1，不成立输出0；输出是判断标志，不是把输入缩放成该
      | 常数。
      |
      | 这里识别一种指令编码。判断成立只说明指令匹配；父级还会结合有效帧、当前模式或其他允许条件决
      | 定是否更新。实际驱动要继续经过控制与板级输出，不能把1理解为硬件执行回执。
  note: ShouDongJian
      | ShouDongJian：只判断一个条件
      |
      | 把输入与5比较，使用关系“==”。成立输出1，不成立输出0；输出是判断标志，不是把输入缩放成该
      | 常数。
      |
      | 这里识别一种指令编码。判断成立只说明指令匹配；父级还会结合有效帧、当前模式或其他允许条件决
      | 定是否更新。实际驱动要继续经过控制与板级输出，不能把1理解为硬件执行回执。
  note: ShouDongYinQi
      | ShouDongYinQi：只判断一个条件
      |
      | 把输入与14比较，使用关系“==”。成立输出1，不成立输出0；输出是判断标志，不是把输入缩放成该
      | 常数。
      |
      | 这里识别一种指令编码。判断成立只说明指令匹配；父级还会结合有效帧、当前模式或其他允许条件决
      | 定是否更新。实际驱动要继续经过控制与板级输出，不能把1理解为硬件执行回执。
  note: ShouDongYouMen
      | ShouDongYouMen：只判断一个条件
      |
      | 把输入与8比较，使用关系“==”。成立输出1，不成立输出0；输出是判断标志，不是把输入缩放成该
      | 常数。
      |
      | 这里识别一种指令编码。判断成立只说明指令匹配；父级还会结合有效帧、当前模式或其他允许条件决
      | 定是否更新。实际驱动要继续经过控制与板级输出，不能把1理解为硬件执行回执。
  note: ShouDongZhuFa
      | ShouDongZhuFa：只判断一个条件
      |
      | 把输入与11比较，使用关系“==”。成立输出1，不成立输出0；输出是判断标志，不是把输入缩放成该
      | 常数。
      |
      | 这里识别一种指令编码。判断成立只说明指令匹配；父级还会结合有效帧、当前模式或其他允许条件决
      | 定是否更新。实际驱动要继续经过控制与板级输出，不能把1理解为硬件执行回执。
  S_Instr : Inport
      settings: AttributesFormatString=S_Instr（指令）
  Logical Operator : Logic  Operator=OR  Inputs=8  AllPortsSameDT=off  OutDataTypeStr=boolean
      settings: AttributesFormatString=Logical Operator（逻辑运算）
  ShouDongBeiFa : simulink/Logic and Bit Operations/Compare To Constant  Description=|  relop===  const=PG_Instr_EblastSet  OutDataTypeStr=boolean
      | ShouDongBeiFa：只判断一个条件
      | 
      | 把输入与12比较，使用关系“==”。成立输出1，不成立输出0；输出是判断标志，不是把输入缩放成该常数。
      | 
      | 这里识别一种指令编码。判断成立只说明指令匹配；父级还会结合有效帧、当前模式或其他允许条件决定是否更新。实际驱动要继续经过控制与板级输出，不能把1理解为硬件执行回执。
      settings: AttributesFormatString=ShouDongBeiFa（手动副阀）
  ShouDongDianHuo : simulink/Logic and Bit Operations/Compare To Constant  Description=|  relop===  const=PG_Instr_FireWorkSet  OutDataTypeStr=boolean
      | ShouDongDianHuo：只判断一个条件
      | 
      | 把输入与10比较，使用关系“==”。成立输出1，不成立输出0；输出是判断标志，不是把输入缩放成该常数。
      | 
      | 这里识别一种指令编码。判断成立只说明指令匹配；父级还会结合有效帧、当前模式或其他允许条件决定是否更新。实际驱动要继续经过控制与板级输出，不能把1理解为硬件执行回执。
      settings: AttributesFormatString=ShouDongDianHuo（手动点火）
  ShouDongDianJi : simulink/Logic and Bit Operations/Compare To Constant  Description=|  relop===  const=PG_Instr_MotorSet  OutDataTypeStr=boolean
      | ShouDongDianJi：只判断一个条件
      | 
      | 把输入与13比较，使用关系“==”。成立输出1，不成立输出0；输出是判断标志，不是把输入缩放成该常数。
      | 
      | 这里识别一种指令编码。判断成立只说明指令匹配；父级还会结合有效帧、当前模式或其他允许条件决定是否更新。实际驱动要继续经过控制与板级输出，不能把1理解为硬件执行回执。
      settings: AttributesFormatString=ShouDongDianJi（手动电机）
  ShouDongJia : simulink/Logic and Bit Operations/Compare To Constant  Description=|  relop===  const=PG_Instr_ManualPlus  OutDataTypeStr=boolean
      | ShouDongJia：只判断一个条件
      | 
      | 把输入与4比较，使用关系“==”。成立输出1，不成立输出0；输出是判断标志，不是把输入缩放成该常数。
      | 
      | 这里识别一种指令编码。判断成立只说明指令匹配；父级还会结合有效帧、当前模式或其他允许条件决定是否更新。实际驱动要继续经过控制与板级输出，不能把1理解为硬件执行回执。
      settings: AttributesFormatString=ShouDongJia（手动增加）
  ShouDongJian : simulink/Logic and Bit Operations/Compare To Constant  Description=|  relop===  const=PG_Instr_ManualrReduce  OutDataTypeStr=boolean
      | ShouDongJian：只判断一个条件
      | 
      | 把输入与5比较，使用关系“==”。成立输出1，不成立输出0；输出是判断标志，不是把输入缩放成该常数。
      | 
      | 这里识别一种指令编码。判断成立只说明指令匹配；父级还会结合有效帧、当前模式或其他允许条件决定是否更新。实际驱动要继续经过控制与板级输出，不能把1理解为硬件执行回执。
      settings: AttributesFormatString=ShouDongJian（手动减小）
  ShouDongYinQi : simulink/Logic and Bit Operations/Compare To Constant  Description=|  relop===  const=PG_Instr_BleedAirSet  OutDataTypeStr=boolean
      | ShouDongYinQi：只判断一个条件
      | 
      | 把输入与14比较，使用关系“==”。成立输出1，不成立输出0；输出是判断标志，不是把输入缩放成该常数。
      | 
      | 这里识别一种指令编码。判断成立只说明指令匹配；父级还会结合有效帧、当前模式或其他允许条件决定是否更新。实际驱动要继续经过控制与板级输出，不能把1理解为硬件执行回执。
      settings: AttributesFormatString=ShouDongYinQi（手动引气）
  ShouDongYouMen : simulink/Logic and Bit Operations/Compare To Constant  Description=|  relop===  const=PG_Instr_OilSet  OutDataTypeStr=boolean
      | ShouDongYouMen：只判断一个条件
      | 
      | 把输入与8比较，使用关系“==”。成立输出1，不成立输出0；输出是判断标志，不是把输入缩放成该常数。
      | 
      | 这里识别一种指令编码。判断成立只说明指令匹配；父级还会结合有效帧、当前模式或其他允许条件决定是否更新。实际驱动要继续经过控制与板级输出，不能把1理解为硬件执行回执。
      settings: AttributesFormatString=ShouDongYouMen（手动油门）
  ShouDongZhuFa : simulink/Logic and Bit Operations/Compare To Constant  Description=|  relop===  const=PG_Instr_EValveSet  OutDataTypeStr=boolean
      | ShouDongZhuFa：只判断一个条件
      | 
      | 把输入与11比较，使用关系“==”。成立输出1，不成立输出0；输出是判断标志，不是把输入缩放成该常数。
      | 
      | 这里识别一种指令编码。判断成立只说明指令匹配；父级还会结合有效帧、当前模式或其他允许条件决定是否更新。实际驱动要继续经过控制与板级输出，不能把1理解为硬件执行回执。
      settings: AttributesFormatString=ShouDongZhuFa（手动主阀）
  S_Start2Manual : Outport
      settings: AttributesFormatString=S_Start2Manual（起动转手动）
  S_Clp2Manual : Outport  Port=2
      settings: AttributesFormatString=S_Clp2Manual（闭环转手动）
  S_Origin2Manual : Outport  Port=3
      settings: AttributesFormatString=S_Origin2Manual（原位转手动）
  wires:
  S_Instr/1 -> ShouDongYinQi/1, ShouDongDianJi/1, ShouDongBeiFa/1, ShouDongZhuFa/1, ShouDongDianHuo/1, ShouDongYouMen/1, ShouDongJian/1, ShouDongJia/1
  ShouDongJia/1 -> Logical Operator/1
  ShouDongJian/1 -> Logical Operator/2
  Logical Operator/1 -> S_Start2Manual/1, S_Origin2Manual/1, S_Clp2Manual/1
  ShouDongYouMen/1 -> Logical Operator/3
  ShouDongDianHuo/1 -> Logical Operator/4
  ShouDongZhuFa/1 -> Logical Operator/5
  ShouDongBeiFa/1 -> Logical Operator/6
  ShouDongDianJi/1 -> Logical Operator/7
  ShouDongYinQi/1 -> Logical Operator/8

== system turbo_controller/FPM/Subsystem/Flag_ECUReset_Reset ==
  note: 在被触发且允许时提出恢复记录清除请求
      |
      | 这是带触发和使能的动作子系统。只有父级满足执行条件时，内部常量1才输出为清除请求；不是模型
      | 每拍都无条件清除FRAM。
      |
      | 本处不发送SPI、不擦除整片存储器，只生成逻辑标志。父级将它与模式变化等条件组合，再由FRAM事
      | 务层决定实际记录处理。
  Enable : EnablePort  StatesWhenEnabling=reset
      settings: AttributesFormatString=Enable（使能）
  Trigger : TriggerPort  TriggerType=falling  VariantControl=(inherit)
      settings: AttributesFormatString=Trigger（触发）
  dth = T0-288.5 : Constant  OutDataTypeStr=uint8  SampleTime=-1
      settings: AttributesFormatString=dth = T0-288.5（固定常量1（旧名称不参与计算））
  S_Flag_ECUReset_Clear : Outport  OutputWhenDisabled=reset  InitialOutput=0
      settings: AttributesFormatString=S_Flag_ECUReset_Clear（清除复位恢复状态请求）
  wires:
  dth = T0-288.5/1 -> S_Flag_ECUReset_Clear/1

== system turbo_controller/BoardInput_输入换算与协议解析/In01_Host（上位机命令解析）/Receive（逐字节组帧与保持有效结果）_108/Step01_取字节与循环控制 ==
  note: 第一步：从本批数据中逐个取字节，决定何时结束循环
      |
      | Rx是最多64项的接收数组，Count说明其中前几项是本次新收到的字节。Index是外面Loop提供的当前序
      | 号，从1开始；它不是已经收到的帧长度。
      |
      | 1. 当前字节=Rx(Index)。Index≤Count时，本字节有效；否则只执行保持，不把数组尾部的旧值当作
      | 新字节。
      | 2. Index≥Count，或者Index=64，任一成立就输出“本批处理结束”。前者表示本批有效字节用完，
      | 后者防止超出64项。
      | 3. 尚未结束时输出下一序号Index+1；结束时输出65，让Loop退出。
      |
      | 例如Count=3，依次处理数组第1、2、3项；到第3项就结束，不再把第4项作为新数据。Count=0时仍会
      | 有一次无效项处理，用于保持命令和处理通知，但不会往帧里加入字节。
      |
      | 本步骤只负责遍历接收数组；它不判断AA55帧头，不校验，不保存命令。Byte和Active送第二步，Last
      | 送第五步，NextIndex反馈Loop。
  接收缓冲_最多64字节 : Inport
  本批有效字节数 : Inport  Port=2
  当前循环序号 : Inport  Port=3
  Active（本项在有效范围内）_15 : RelationalOperator  Operator=<=  OutDataTypeStr=boolean  RndMeth=Simplest  InputSameDT=off
  Add（加减运算）_22 : Sum  SaturateOnIntegerOverflow=on  OutDataTypeStr=Inherit: Same as first input
  AtLimit（达到处理上限）_18 : RelationalOperator  Operator===  OutDataTypeStr=boolean  RndMeth=Simplest  InputSameDT=off
  Constant（常量）_17 : Constant  Value=64  OutDataTypeStr=uint32
  Constant（常量）_20 : Constant  Value=65  OutDataTypeStr=uint32
  Constant（常量）_21 : Constant  OutDataTypeStr=uint32
  CurrentByte（按接收顺序取字节）_24 : Selector  InputPortWidth=64  IndexOptions=Index vector (port)  Indices=1  OutputSizes=1
  Last（本周期最后一项）_19 : Logic  Operator=OR  IconShape=distinctive  AllPortsSameDT=off  OutDataTypeStr=boolean
  NextIndex（处理下一项或结束）_23 : Switch  Criteria=u2 ~= 0  SaturateOnIntegerOverflow=off  InputSameDT=off
  ReceivedAll（已处理所有有效项）_16 : RelationalOperator  OutDataTypeStr=boolean  RndMeth=Simplest  InputSameDT=off
  当前字节 : Outport
  本字节有效 : Outport  Port=2
  本批处理结束 : Outport  Port=3
  下一循环序号 : Outport  Port=4
  wires:
  NextIndex（处理下一项或结束）_23/1 -> 下一循环序号/1
  Active（本项在有效范围内）_15/1 -> 本字节有效/1
  CurrentByte（按接收顺序取字节）_24/1 -> 当前字节/1
  接收缓冲_最多64字节/1 -> CurrentByte（按接收顺序取字节）_24/1
  Add（加减运算）_22/1 -> NextIndex（处理下一项或结束）_23/3
  Last（本周期最后一项）_19/1 -> NextIndex（处理下一项或结束）_23/2, 本批处理结束/1
  Constant（常量）_20/1 -> NextIndex（处理下一项或结束）_23/1
  Constant（常量）_21/1 -> Add（加减运算）_22/2
  AtLimit（达到处理上限）_18/1 -> Last（本周期最后一项）_19/2
  ReceivedAll（已处理所有有效项）_16/1 -> Last（本周期最后一项）_19/1
  Constant（常量）_17/1 -> AtLimit（达到处理上限）_18/2
  本批有效字节数/1 -> ReceivedAll（已处理所有有效项）_16/2, Active（本项在有效范围内）_15/2
  当前循环序号/1 -> Add（加减运算）_22/1, CurrentByte（按接收顺序取字节）_24/2, Active（本项在有效范围内）_15/1, ReceivedAll（已处理所有有效项）_16/1, AtLimit（达到处理上限）_18/1

== system turbo_controller/BoardInput_输入换算与协议解析/In01_Host（上位机命令解析）/Receive（逐字节组帧与保持有效结果）_108/Step02_拼帧并记住未收完的数据 ==
  note: 第二步：识别帧头、拼满14字节，并记住半帧
      |
      | 输入是一项字节及“本字节有效”标志。内部Collect按AA、55识别帧头，接着按顺序把后续字节放进1
      | 4项候选缓存，收齐时给出Complete。
      |
      | Buffer保存尚未验证的候选内容，Position保存下一项要放的位置。每个字节处理后，新的缓存与位置
      | 经过类型转换存回记忆，供下一个字节使用；本批结束时也不清掉，因此可跨接收批次续收。
      |
      | 例：第一次只收到AA、55及其后6字节，第二次又收到剩余6字节，第二次会继续原位置，直到拼满14字
      | 节。无效项不会推进收帧。
      |
      | 输出“候选帧”只是凑齐的内容，尚不能当命令使用；输出“本字节刚好收齐”是一次完成事件。两者
      | 送第三步校验，候选内容也送第四步等待是否接受。
      |
      | 这里的延迟按循环处理的节奏保存记忆，不是在每个字节之间额外等待1 ms。更细的帧头重同步规则仍
      | 在Collect内部，原逻辑未改。
  当前字节 : Inport
  本字节有效 : Inport  Port=2
  Buffer（跨周期收帧缓存）_25 : UnitDelay  InitialCondition=uint8(zeros(14,1))  SampleTime=-1  HasFrameUpgradeWarning=on
  Collect（帧头识别与缓存推进）_66 : Subsystem  Description=|
      | 逐字节组帧：本页只做“找帧头、存字节、推进位置”
      | 
      | 固定帧长为14字节，帧头是十六进制AA、55。输入为上一份候选缓存、已收字节数Position、本次Byte和本字节有效Active。输出为更新缓存、下一次使用的Position和本次收齐事件Complete。
      | 
      | Position不是本批接收数组的序号：0表示还在找AA，1表示已见AA、正在等55，2～13表示头部已确认、继续收后面的内容。跨调用的记忆由外层Step02保存，本页根据输入计算一次更新。
      | 
      | 按五步看：
      | 1 判断当前是否在等AA或55，以及字节是否匹配。
      | 2 决定这个字节应不应该进入候选缓存。
      | 3 算出本次写入位置Position+1，判断是否达到14。
      | 4 允许写入才更新对应一项，否则保留原缓存。
      | 5 按找头、重同步、收齐和无效字节规则，决定下一位置及Complete。
      | 
      | 例：AA→AA→55时，第二个AA保留继续等55的机会，不当作第二帧头写入；头确认后，后续数据即使也是AA或55，仍按普通数据收下。无效字节不推进位置，也不发收齐事件。
      | 
      | Complete仅表示候选帧刚拼满，不表示校验通过；外面的校验步骤还会检查内容。这里没有重写协议或增加等待时间，五步在同一次字节处理内完成。
  Position（已收到的字节数）_26 : UnitDelay  InitialCondition=uint16(0)  SampleTime=-1  HasFrameUpgradeWarning=on
  Store_uint16（按十六位无符号数保存状态）_536487 : DataTypeConversion  Description=为反馈回路显式指定原程序的状态类型，保持原状态更新节拍。  OutDataTypeStr=uint16  RndMeth=Round
  Store_uint8（按八位无符号数保存状态）_536486 : DataTypeConversion  Description=为反馈回路显式指定原程序的状态类型，保持原状态更新节拍。  OutDataTypeStr=uint8  RndMeth=Round
  候选14字节帧 : Outport
  本字节刚好收齐 : Outport  Port=2
  wires:
  Collect（帧头识别与缓存推进）_66/3(Complete（本字节组成完整帧）_65) -> 本字节刚好收齐/1  "Collect（帧头识别与缓存推进）"
  Collect（帧头识别与缓存推进）_66/2(Position（下次接收位置）_64) -> Store_uint16（按十六位无符号数保存状态）_536487/1  "Collect（帧头识别与缓存推进）"
  Collect（帧头识别与缓存推进）_66/1(Buffer（更新后的帧缓存）_63) -> 候选14字节帧/1, Store_uint8（按八位无符号数保存状态）_536486/1  "Collect（帧头识别与缓存推进）"
  本字节有效/1 -> Collect（帧头识别与缓存推进）_66/4(Active（当前字节有效）_30)
  当前字节/1 -> Collect（帧头识别与缓存推进）_66/3(Byte（当前字节）_29)
  Position（已收到的字节数）_26/1 -> Collect（帧头识别与缓存推进）_66/2(Position（已收字节数）_28)
  Buffer（跨周期收帧缓存）_25/1 -> Collect（帧头识别与缓存推进）_66/1(Buffer（上次收帧缓存）_27)
  Store_uint16（按十六位无符号数保存状态）_536487/1 -> Position（已收到的字节数）_26/1
  Store_uint8（按八位无符号数保存状态）_536486/1 -> Buffer（跨周期收帧缓存）_25/1

== system turbo_controller/BoardInput_输入换算与协议解析/In01_Host（上位机命令解析）/Receive（逐字节组帧与保持有效结果）_108/Step03_检查完整性与双校验 ==
  note: 第三步：这一帧既要收齐，也要两种校验都通过
      |
      | Verify只对已收齐的14字节候选帧作有效性检查。对第1～12字节重新计算：
      | 累加校验=这12字节之和 mod 256；
      | 异或校验=第1字节 XOR 第2字节 XOR … XOR 第12字节。
      | 分别与第13、第14字节比较，两项均匹配才通过。
      |
      | 最终接受事件=“本字节刚好收齐” AND “Verify通过”。即使Verify保留着上一帧的通过状态，没有
      | 本次Complete也不会再次接受旧内容。
      |
      | 例如数据未收满、累加校验不符、异或校验不符，任意一种都会使本次接受事件为假。为真时通知第四
      | 步更新命令，并通知第五步记住有新命令待报告。
      |
      | 本处检查的是通信内容是否符合校验，不判断某条起动命令在当前发动机状态下是否允许执行；命令解
      | 释与模式判断在后面的CMMRead、ESM。
  本字节刚好收齐 : Inport
  候选14字节帧 : Inport  Port=2
  Accepted（本字节完成一帧有效数据）_94 : Logic  IconShape=distinctive  AllPortsSameDT=off  OutDataTypeStr=boolean
  Cast（数据类型转换）_92 : DataTypeConversion  OutDataTypeStr=uint32  RndMeth=Round
  Verify（完整帧校验）_93 : Subsystem  Description=|
      | 上位机候选帧怎样通过最后检查
      | 
      | Collect已经收齐14字节后，本模块才开始检查。Complete转成0或1次的执行许可：不完整时不重新计算，以免读到半帧；完整时取协议规定的数据段，同时计算累加与异或校验。
      | 
      | Checksum中两种规则分别为：
      | 累加校验 = 所有待校验字节之和对256取余；
      | 异或校验 = 所有待校验字节逐个按位异或。
      | 计算出的两项分别与候选帧尾部校验项比较，两项都相同才输出通过。
      | 
      | 校验失败时，外层Receive保留旧命令，等待下一帧。外层还把“校验通过”和“本次刚收齐”组合，避免把上次通过的保持值误当成本次新帧也通过。
      | 
      | 这里不解释FC、F0等命令含义；命令解码要等数据可靠之后交给CMMRead/Instr_Analyse。
      | 
      | 本实例对第1～12字节计算累加和及异或值，分别与第13、第14字节比较。
  本字节接受新命令 : Outport
  wires:
  Accepted（本字节完成一帧有效数据）_94/1 -> 本字节接受新命令/1
  Verify（完整帧校验）_93/1(Valid（校验是否通过）_91) -> Accepted（本字节完成一帧有效数据）_94/2  "Verify（完整帧校验）"
  候选14字节帧/1 -> Verify（完整帧校验）_93/2(Frame（完整候选帧）_69)
  Cast（数据类型转换）_92/1 -> Verify（完整帧校验）_93/1(Complete（完整帧执行一次）_67)
  本字节刚好收齐/1 -> Cast（数据类型转换）_92/1, Accepted（本字节完成一帧有效数据）_94/1

== system turbo_controller/BoardInput_输入换算与协议解析/In01_Host（上位机命令解析）/Receive（逐字节组帧与保持有效结果）_108/Step04_只保存通过校验的命令 ==
  note: 第四步：只用有效帧更新命令，坏帧不能覆盖好命令
      |
      | 将14字节候选帧后面补36个0，保持原工程50项命令接口：前14项是收到的帧，15～50项为兼容占位。
      |
      | 本次接受事件为真：选择这组新命令，并存入Latest；
      | 本次接受事件为假：继续输出Latest记住的旧命令。
      |
      | 例如上一条有效命令是A，本批又来了校验错误的B，输出仍为A；B不会因为已经凑满14字节就覆盖A。
      | 首次尚未接受命令时，沿用原有初始值。
      |
      | 一个接收批次可能连续有多条有效帧，每接受一条就更新一次，批次结束后输出最后一条。这个50项数
      | 组是最近有效结果，不是每次通知就自动清空的队列。
      |
      | 输出交外层Command。是否让控制任务在本拍使用它，由第五步的通知Flag另行表示。
  本字节接受新命令 : Inport
  候选14字节帧 : Inport  Port=2
  Latest（最近有效上位机命令）_95 : UnitDelay  InitialCondition=uint8(zeros(50,1))  SampleTime=-1  HasFrameUpgradeWarning=on
  Pack（按顺序拼接）_98 : Mux  Inputs=2
  Padding（补齐五十字节命令接口）_97 : Constant  Value=zeros(36,1)  OutDataTypeStr=uint8
  Store_uint8（按八位无符号数保存状态）_536492 : DataTypeConversion  Description=为反馈回路显式指定原程序的状态类型，保持原状态更新节拍。  OutDataTypeStr=uint8  RndMeth=Round
  UpdateCommand（有效帧才更新命令）_99 : Switch  Criteria=u2 ~= 0  SaturateOnIntegerOverflow=off  InputSameDT=off
  最近有效命令_50字节 : Outport
  wires:
  UpdateCommand（有效帧才更新命令）_99/1 -> 最近有效命令_50字节/1, Store_uint8（按八位无符号数保存状态）_536492/1
  Latest（最近有效上位机命令）_95/1 -> UpdateCommand（有效帧才更新命令）_99/3
  本字节接受新命令/1 -> UpdateCommand（有效帧才更新命令）_99/2
  Pack（按顺序拼接）_98/1 -> UpdateCommand（有效帧才更新命令）_99/1
  Padding（补齐五十字节命令接口）_97/1 -> Pack（按顺序拼接）_98/2
  候选14字节帧/1 -> Pack（按顺序拼接）_98/1
  Store_uint8（按八位无符号数保存状态）_536492/1 -> Latest（最近有效上位机命令）_95/1

== system turbo_controller/BoardInput_输入换算与协议解析/In01_Host（上位机命令解析）/Receive（逐字节组帧与保持有效结果）_108/Step05_等到20毫秒再通知一次 ==
  note: 第五步：记住新命令，等20 ms更新时机再通知
      |
      | Accepted表示本字节刚接受了有效帧，Fresh表示以前收到了有效帧但尚未报告。两者用OR合成NewSeen
      | ：只要其中一个为真，就说明有新命令等着通知。
      |
      | 输出Flag=ControlTick AND NewSeen，再转成原接口数据类型。ControlTick由外层给出，表示当前到
      | 了20 ms更新时机；本步骤自己不计时，也不把秒数当输入。
      |
      | 记忆更新：只有“本批处理结束 AND ControlTick”同时成立，才把待通知标志清零；其余时候继续保
      | 存NewSeen。这样循环尚未处理完时不会过早丢掉通知。
      |
      | 例：第5 ms收到了有效帧，命令先被第四步保存，待通知状态保持；第20 ms更新许可到来时给出Flag
      | ，批次处理结束后清除。若这期间没有新帧，第40 ms不会再通知一次。
      |
      | 同一更新间隔内收到多帧，通知表示“有更新”，第四步给出最近一条，不为每一帧单独排队。Flag是
      | 给控制任务的通知，不是向上位机发送的应答。
  本字节接受新命令 : Inport
  本批处理结束 : Inport  Port=2
  20毫秒更新许可 : Inport  Port=3
  Cast（数据类型转换）_105 : DataTypeConversion  OutDataTypeStr=uint8  RndMeth=Round
  ClearAfterReport（20毫秒报告后清标志）_103 : Switch  Criteria=u2 ~= 0  SaturateOnIntegerOverflow=off  InputSameDT=off
  Condition（条件组合）_104 : Logic  IconShape=distinctive  AllPortsSameDT=off  OutDataTypeStr=boolean
  Constant（常量）_102 : Constant  Value=false  OutDataTypeStr=boolean
  Fresh（尚未报告的新命令）_96 : UnitDelay  InitialCondition=logical(0)  SampleTime=-1  HasFrameUpgradeWarning=on
  NewSeen（存在未报告的新命令）_100 : Logic  Operator=OR  IconShape=distinctive  AllPortsSameDT=off  OutDataTypeStr=boolean
  ReportDone（本周期处理完并报告）_101 : Logic  IconShape=distinctive  AllPortsSameDT=off  OutDataTypeStr=boolean
  Store_boolean（按逻辑值保存状态）_536493 : DataTypeConversion  Description=为反馈回路显式指定原程序的状态类型，保持原状态更新节拍。  OutDataTypeStr=boolean  RndMeth=Round
  新命令通知 : Outport
  wires:
  Cast（数据类型转换）_105/1 -> 新命令通知/1
  ClearAfterReport（20毫秒报告后清标志）_103/1 -> Store_boolean（按逻辑值保存状态）_536493/1
  Condition（条件组合）_104/1 -> Cast（数据类型转换）_105/1
  NewSeen（存在未报告的新命令）_100/1 -> ClearAfterReport（20毫秒报告后清标志）_103/3, Condition（条件组合）_104/2
  ReportDone（本周期处理完并报告）_101/1 -> ClearAfterReport（20毫秒报告后清标志）_103/2
  Constant（常量）_102/1 -> ClearAfterReport（20毫秒报告后清标志）_103/1
  20毫秒更新许可/1 -> Condition（条件组合）_104/1, ReportDone（本周期处理完并报告）_101/2
  本批处理结束/1 -> ReportDone（本周期处理完并报告）_101/1
  本字节接受新命令/1 -> NewSeen（存在未报告的新命令）_100/2
  Fresh（尚未报告的新命令）_96/1 -> NewSeen（存在未报告的新命令）_100/1
  Store_boolean（按逻辑值保存状态）_536493/1 -> Fresh（尚未报告的新命令）_96/1

== system turbo_controller/BoardInput_输入换算与协议解析/In02_Motor（电机反馈解析）/Receive（逐字节组帧与保持有效结果）_235/Step01_取字节与循环控制 ==
  note: 第一步：只处理本批收到的字节
      |
      | 接收数组最多64项，Count是这次新收到的数量，Loop给出从1开始的Index。Byte=Rx(Index)，Active=
      | (Index≤Count)。
      |
      | 处理到Index≥Count或Index=64，就把下一循环序号设65，使Loop退出；否则下一序号=Index+1。Coun
      | t=3只处理第1～3项；Count=0时仍走一次无效项保持路径，但不会把数组旧值加入帧。
      |
      | 输出Byte和Active给组帧步骤，下一序号反馈Loop。这里不识别帧头，不作CRC，不把Index当作跨批收
      | 帧位置。
  输入1_本批循环序号 : Inport
  输入2_本批有效字节数 : Inport  Port=2
  输入3_本批接收数组 : Inport  Port=3
  Active（本项在有效范围内）_116 : RelationalOperator  Operator=<=  OutDataTypeStr=boolean  RndMeth=Simplest  InputSameDT=off
  Add（加减运算）_123 : Sum  SaturateOnIntegerOverflow=on  OutDataTypeStr=Inherit: Same as first input
  AtLimit（达到处理上限）_119 : RelationalOperator  Operator===  OutDataTypeStr=boolean  RndMeth=Simplest  InputSameDT=off
  Constant（常量）_118 : Constant  Value=64  OutDataTypeStr=uint32
  Constant（常量）_121 : Constant  Value=65  OutDataTypeStr=uint32
  Constant（常量）_122 : Constant  OutDataTypeStr=uint32
  CurrentByte（按接收顺序取字节）_125 : Selector  InputPortWidth=64  IndexOptions=Index vector (port)  Indices=1  OutputSizes=1
  Last（本周期最后一项）_120 : Logic  Operator=OR  IconShape=distinctive  AllPortsSameDT=off  OutDataTypeStr=boolean
  NextIndex（处理下一项或结束）_124 : Switch  Criteria=u2 ~= 0  SaturateOnIntegerOverflow=off  InputSameDT=off
  ReceivedAll（已处理所有有效项）_117 : RelationalOperator  OutDataTypeStr=boolean  RndMeth=Simplest  InputSameDT=off
  输出1_本项字节 : Outport
  输出2_本项字节有效 : Outport  Port=2
  输出3_下一循环序号 : Outport  Port=3
  wires:
  NextIndex（处理下一项或结束）_124/1 -> 输出3_下一循环序号/1
  Active（本项在有效范围内）_116/1 -> 输出2_本项字节有效/1
  CurrentByte（按接收顺序取字节）_125/1 -> 输出1_本项字节/1
  Add（加减运算）_123/1 -> NextIndex（处理下一项或结束）_124/3
  Last（本周期最后一项）_120/1 -> NextIndex（处理下一项或结束）_124/2
  Constant（常量）_121/1 -> NextIndex（处理下一项或结束）_124/1
  AtLimit（达到处理上限）_119/1 -> Last（本周期最后一项）_120/2
  ReceivedAll（已处理所有有效项）_117/1 -> Last（本周期最后一项）_120/1
  输入3_本批接收数组/1 -> CurrentByte（按接收顺序取字节）_125/1
  Constant（常量）_118/1 -> AtLimit（达到处理上限）_119/2
  Constant（常量）_122/1 -> Add（加减运算）_123/2
  输入2_本批有效字节数/1 -> ReceivedAll（已处理所有有效项）_117/2, Active（本项在有效范围内）_116/2
  输入1_本批循环序号/1 -> Add（加减运算）_123/1, ReceivedAll（已处理所有有效项）_117/1, Active（本项在有效范围内）_116/1, AtLimit（达到处理上限）_119/1, CurrentByte（按接收顺序取字节）_125/2

== system turbo_controller/BoardInput_输入换算与协议解析/In02_Motor（电机反馈解析）/Receive（逐字节组帧与保持有效结果）_235/Step02_拼帧并保存半帧 ==
  note: 第二步：跨多次接收保存半帧
      |
      | 将本项字节、有效标志、上次候选缓存和上次收帧Position交给Collect。Collect识别AA55并逐项填满
      | 9字节，具体规则已在其内部再拆成五步。
      |
      | 更新后的缓存和Position经原数据类型转换，送回两条记忆块；所以第一次只收到一半，下一批还能接
      | 着填，不必从头找AA。输出候选帧与“本字节刚收齐”，交第三步校验。
      |
      | 候选缓存不等于已接受结果。即使旧缓存里已经有完整内容，没有本次收齐事件也不能再次接受它。这
      | 里的记忆按原循环节奏推进，没有增加一个额外的采样周期等待。
  输入1_本项字节 : Inport
  输入2_本项字节有效 : Inport  Port=2
  Buffer（跨周期收帧缓存）_126 : UnitDelay  InitialCondition=uint8(zeros(9,1))  SampleTime=-1  HasFrameUpgradeWarning=on
  Collect（帧头识别与缓存推进）_167 : Subsystem  Description=|
      | 逐字节组帧：本页只做“找帧头、存字节、推进位置”
      | 
      | 固定帧长为9字节，帧头是十六进制AA、55。输入为上一份候选缓存、已收字节数Position、本次Byte和本字节有效Active。输出为更新缓存、下一次使用的Position和本次收齐事件Complete。
      | 
      | Position不是本批接收数组的序号：0表示还在找AA，1表示已见AA、正在等55，2～8表示头部已确认、继续收后面的内容。跨调用的记忆由外层Step02保存，本页根据输入计算一次更新。
      | 
      | 按五步看：
      | 1 判断当前是否在等AA或55，以及字节是否匹配。
      | 2 决定这个字节应不应该进入候选缓存。
      | 3 算出本次写入位置Position+1，判断是否达到9。
      | 4 允许写入才更新对应一项，否则保留原缓存。
      | 5 按找头、重同步、收齐和无效字节规则，决定下一位置及Complete。
      | 
      | 例：AA→AA→55时，第二个AA保留继续等55的机会，不当作第二帧头写入；头确认后，后续数据即使也是AA或55，仍按普通数据收下。无效字节不推进位置，也不发收齐事件。
      | 
      | Complete仅表示候选帧刚拼满，不表示校验通过；外面的校验步骤还会检查内容。这里没有重写协议或增加等待时间，五步在同一次字节处理内完成。
  Position（已收到的字节数）_127 : UnitDelay  InitialCondition=uint16(0)  SampleTime=-1  HasFrameUpgradeWarning=on
  Store_uint16（按十六位无符号数保存状态）_536588 : DataTypeConversion  Description=为反馈回路显式指定原程序的状态类型，保持原状态更新节拍。  OutDataTypeStr=uint16  RndMeth=Round
  Store_uint8（按八位无符号数保存状态）_536587 : DataTypeConversion  Description=为反馈回路显式指定原程序的状态类型，保持原状态更新节拍。  OutDataTypeStr=uint8  RndMeth=Round
  输出1_本字节刚收齐 : Outport
  输出2_候选帧缓存 : Outport  Port=2
  wires:
  Collect（帧头识别与缓存推进）_167/3(Complete（本字节组成完整帧）_166) -> 输出1_本字节刚收齐/1  "Collect（帧头识别与缓存推进）"
  Collect（帧头识别与缓存推进）_167/1(Buffer（更新后的帧缓存）_164) -> Store_uint8（按八位无符号数保存状态）_536587/1, 输出2_候选帧缓存/1  "Collect（帧头识别与缓存推进）"
  Collect（帧头识别与缓存推进）_167/2(Position（下次接收位置）_165) -> Store_uint16（按十六位无符号数保存状态）_536588/1  "Collect（帧头识别与缓存推进）"
  Store_uint16（按十六位无符号数保存状态）_536588/1 -> Position（已收到的字节数）_127/1
  输入2_本项字节有效/1 -> Collect（帧头识别与缓存推进）_167/4(Active（当前字节有效）_131)
  输入1_本项字节/1 -> Collect（帧头识别与缓存推进）_167/3(Byte（当前字节）_130)
  Position（已收到的字节数）_127/1 -> Collect（帧头识别与缓存推进）_167/2(Position（已收字节数）_129)
  Buffer（跨周期收帧缓存）_126/1 -> Collect（帧头识别与缓存推进）_167/1(Buffer（上次收帧缓存）_128)
  Store_uint8（按八位无符号数保存状态）_536587/1 -> Buffer（跨周期收帧缓存）_126/1

== system turbo_controller/BoardInput_输入换算与协议解析/In02_Motor（电机反馈解析）/Receive（逐字节组帧与保持有效结果）_235/Step03_收齐且校验通过才接受 ==
  note: 第三步：刚收齐且CRC通过，才接受新帧
      |
      | Complete表示这一项字节刚把9字节补齐，先按原类型传给Verify触发校验。Verify对第6～7字节计算C
      | RC16，分别与第8、9字节的高、低校验字节比较。
      |
      | 最后Accepted=Complete AND Verify通过。这样未收齐的数据不会被采用，Verify上一帧保留的通过状
      | 态也不会在没有新Complete时重新接收旧帧。
      |
      | CRC初值、表和覆盖范围保留原设置。校验失败只让本次Accepted为假；后面的保持步骤继续输出上一
      | 有效反馈。本处不作反馈比例换算，不直接生成驱动命令。
  输入1_本字节刚收齐 : Inport
  输入2_候选帧缓存 : Inport  Port=2
  Accepted（本字节完成一帧有效数据）_219 : Logic  IconShape=distinctive  AllPortsSameDT=off  OutDataTypeStr=boolean
  Cast（数据类型转换）_217 : DataTypeConversion  OutDataTypeStr=uint32  RndMeth=Round
  Verify（完整帧校验）_218 : Subsystem  Description=|
      | 电机9字节反馈怎样核对CRC
      | 
      | Collect送来的是候选完整帧，本模块只在Complete有效时执行校验。内部取协议指定的待校验字节段，送CRC16逐字节计算，并取出帧尾携带的两个CRC字节。
      | 
      | 16位计算结果分为高低两部分：高字节=floor(CRC/256)，低字节=bitand(CRC,255)。分别与帧中对应位置比较，两项都一致才给出有效结果。
      | 
      | 比如计算CRC为十六进制1234，协议中的CRC高字节必须是12、低字节必须是34；顺序反过来也不能通过。CRC覆盖范围由本页Selector的固定索引决定，不应把帧头或尾部CRC自身随意加入。
      | 
      | 输出交给Receive，与“这一轮确实刚收齐一帧”共同决定是否更新反馈。不完整或校验错误时，外层保留最近有效结果。
      | 
      | 本实例CRC覆盖第6～7字节，接收的CRC高、低字节在第8、9字节。
  输出1_本字节接受有效帧 : Outport
  wires:
  Accepted（本字节完成一帧有效数据）_219/1 -> 输出1_本字节接受有效帧/1
  输入2_候选帧缓存/1 -> Verify（完整帧校验）_218/2(Frame（完整候选帧）_170)
  Cast（数据类型转换）_217/1 -> Verify（完整帧校验）_218/1(Complete（完整帧执行一次）_168)
  Verify（完整帧校验）_218/1(Valid（校验是否通过）_216) -> Accepted（本字节完成一帧有效数据）_219/2  "Verify（完整帧校验）"
  输入1_本字节刚收齐/1 -> Accepted（本字节完成一帧有效数据）_219/1, Cast（数据类型转换）_217/1

== system turbo_controller/BoardInput_输入换算与协议解析/In02_Motor（电机反馈解析）/Receive（逐字节组帧与保持有效结果）_235/Step04_换算反馈并保持有效结果 ==
  note: 第四步：把电机有效帧换算成反馈，并保持结果
      |
      | 取候选帧第6字节为高字节、第7字节为低字节，先转成可运算类型，再计算：
      | 原始整数=第6字节×256+第7字节；
      | 候选反馈=floor(原始整数/3)。
      | 例如高1、低44合成300，除3后输出100。除3与向下取整均沿用原协议。
      |
      | Accepted为真才更新输出和Motor记忆；为假则直接用旧值。坏帧或半帧不会覆盖上一有效反馈，同批
      | 多帧会按字节顺序逐次更新，最终保留最后一条。
      |
      | 输出交外层测速来源选择。本步骤不发送电机命令，也不证明反馈没有超时；来源与超时判断仍在In05
      | _Speed中完成。
  输入1_候选帧缓存 : Inport
  输入2_本字节接受有效帧 : Inport  Port=2
  Cast（数据类型转换）_222 : DataTypeConversion  OutDataTypeStr=uint16  RndMeth=Round
  Cast（数据类型转换）_224 : DataTypeConversion  OutDataTypeStr=uint16  RndMeth=Round
  Cast（数据类型转换）_228 : DataTypeConversion  OutDataTypeStr=double  RndMeth=Round
  Cast（数据类型转换）_232 : DataTypeConversion  OutDataTypeStr=single  RndMeth=Round
  Constant（常量）_225 : Constant  Value=256  OutDataTypeStr=uint16
  Constant（常量）_229 : Constant  Value=3  OutDataTypeStr=double
  Divide（相除）_230 : Product  Inputs=*/  SaturateOnIntegerOverflow=on  OutDataTypeStr=Inherit: Same as first input
  High（原始数值高字节）_221 : Selector  InputPortWidth=9  IndexOptions=Index vector (dialog)  Indices=6  OutputSizes=1
  HoldOrUpdate（无有效帧时保持上次反馈）_233 : Switch  Criteria=u2 ~= 0  SaturateOnIntegerOverflow=off  InputSameDT=off
  Low（原始数值低字节）_223 : Selector  InputPortWidth=9  IndexOptions=Index vector (dialog)  Indices=7  OutputSizes=1
  Motor（保持电机反馈转速）_220 : UnitDelay  InitialCondition=single(0)  SampleTime=-1  HasFrameUpgradeWarning=on
  Multiply（相乘）_226 : Product  Inputs=**  SaturateOnIntegerOverflow=on  OutDataTypeStr=Inherit: Same as first input
  Raw16（合成十六位原始数值）_227 : Sum  SaturateOnIntegerOverflow=on  OutDataTypeStr=Inherit: Same as first input
  Round（取整）_231 : Rounding
  Store_single（按单精度数保存状态）_536593 : DataTypeConversion  Description=为反馈回路显式指定原程序的状态类型，保持原状态更新节拍。  OutDataTypeStr=single  RndMeth=Round
  输出1_最近有效反馈 : Outport
  wires:
  HoldOrUpdate（无有效帧时保持上次反馈）_233/1 -> 输出1_最近有效反馈/1, Store_single（按单精度数保存状态）_536593/1
  Divide（相除）_230/1 -> Round（取整）_231/1
  Cast（数据类型转换）_224/1 -> Raw16（合成十六位原始数值）_227/2
  Multiply（相乘）_226/1 -> Raw16（合成十六位原始数值）_227/1
  Constant（常量）_225/1 -> Multiply（相乘）_226/2
  Cast（数据类型转换）_222/1 -> Multiply（相乘）_226/1
  Store_single（按单精度数保存状态）_536593/1 -> Motor（保持电机反馈转速）_220/1
  Motor（保持电机反馈转速）_220/1 -> HoldOrUpdate（无有效帧时保持上次反馈）_233/3
  输入2_本字节接受有效帧/1 -> HoldOrUpdate（无有效帧时保持上次反馈）_233/2
  Cast（数据类型转换）_232/1 -> HoldOrUpdate（无有效帧时保持上次反馈）_233/1
  输入1_候选帧缓存/1 -> High（原始数值高字节）_221/1, Low（原始数值低字节）_223/1
  Constant（常量）_229/1 -> Divide（相除）_230/2
  Cast（数据类型转换）_228/1 -> Divide（相除）_230/1
  Round（取整）_231/1 -> Cast（数据类型转换）_232/1
  Raw16（合成十六位原始数值）_227/1 -> Cast（数据类型转换）_228/1
  Low（原始数值低字节）_223/1 -> Cast（数据类型转换）_224/1
  High（原始数值高字节）_221/1 -> Cast（数据类型转换）_222/1
